simulink model "Three_Phase_Controlled"  (R2025b)
settings: Solver=VariableStepAuto  StartTime=0.0  StopTime=10.0  MaxStep=1e-4  RelTol=1e-3
libraries: nesl_utility x15, ee_lib x14, fl_lib x10
settings Model: Creator=USER  LastModifiedBy=USER

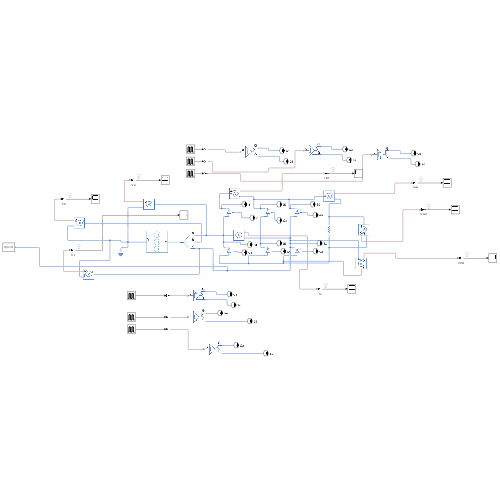
[thumbnail: Simulink's stored preview of the top-level diagram]
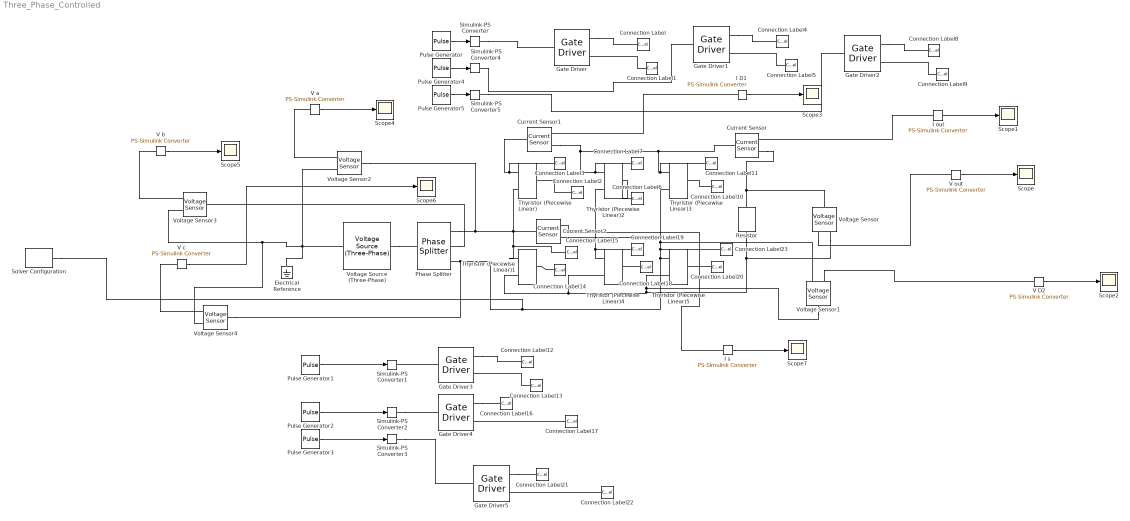
== system Three_Phase_Controlled ==
  Connection Label : ConnectionLabel  Label=G1
  Connection Label1 : ConnectionLabel  Label=S1
  Connection Label10 : ConnectionLabel  Label=G5
  Connection Label11 : ConnectionLabel  Label=S5
  Connection Label12 : ConnectionLabel  Label=G4
  Connection Label13 : ConnectionLabel  Label=S4
  Connection Label14 : ConnectionLabel  Label=G4
  Connection Label15 : ConnectionLabel  Label=S4
  Connection Label16 : ConnectionLabel  Label=G6
  Connection Label17 : ConnectionLabel  Label=S6
  Connection Label18 : ConnectionLabel  Label=G6
  Connection Label19 : ConnectionLabel  Label=S6
  Connection Label2 : ConnectionLabel  Label=G1
  Connection Label20 : ConnectionLabel  Label=G2
  Connection Label21 : ConnectionLabel  Label=G2
  Connection Label22 : ConnectionLabel  Label=S2
  Connection Label23 : ConnectionLabel  Label=S2
  Connection Label3 : ConnectionLabel  Label=S1
  Connection Label4 : ConnectionLabel  Label=G3
  Connection Label5 : ConnectionLabel  Label=S3
  Connection Label6 : ConnectionLabel  Label=G3
  Connection Label7 : ConnectionLabel  Label=S3
  Connection Label8 : ConnectionLabel  Label=G5
  Connection Label9 : ConnectionLabel  Label=S5
  Current Sensor : fl_lib/Electrical/Electrical Sensors/Current Sensor
  Current Sensor1 : fl_lib/Electrical/Electrical Sensors/Current Sensor
  Current Sensor2 : fl_lib/Electrical/Electrical Sensors/Current Sensor
  Electrical Reference : fl_lib/Electrical/Electrical Elements/Electrical Reference
  Gate Driver{,1..5} (6 alike) : ee_lib/Semiconductors & Converters/Gate Driver  port_option=ee.enum.controlport.ps  uHigh=2.0 V  uLow=0.8 V  uHighValue=0.7  uLowValue=0.3  vHigh=15 V  vLow=0 V  tHigh=50 ns  tLow=50 ns  parameterization=ee.enum.semiconductors.gateDriverParam.outputImpedance  rHigh=2 Ohm  rLow=2 Ohm  tRise=20 ns  tFall=20 ns  cLoad=10 nF  ZonTime_specify=off  ZonTime_priority=None  ZonTime=0 s  ZoffTime_specify=off  ZoffTime_priority=None  ZoffTime=0 s
      settings: InternalSimscapePortConfiguration="{\"Bottom\":[],\"Left\":[{\"id\":\"u\",\"label\":\"u\",\"type\":\"input\"}],\"Right\":[{\"id\":\"G\",\"label\":\"G\",\"type\":\"foundation.electrical.electrical\"},{\"id\":\"S\",\"label\":\"S\",\"type\":\"foundation.electrical.electrical\"}],\"Top\":[]}"
  I D1 : nesl_utility/PS-Simulink Converter  PhysicalDomain=network_engine_domain  SubClassName=ps_output  LeftPortType=input  RightPortType=output  PseudoPeriodic=off  Frequencies=[]  VectorFormat=inherit  Unit=inherit  AffineConversion=off
  I out : nesl_utility/PS-Simulink Converter  PhysicalDomain=network_engine_domain  SubClassName=ps_output  LeftPortType=input  RightPortType=output  PseudoPeriodic=off  Frequencies=[]  VectorFormat=inherit  Unit=inherit  AffineConversion=off
  I s : nesl_utility/PS-Simulink Converter  PhysicalDomain=network_engine_domain  SubClassName=ps_output  LeftPortType=input  RightPortType=output  PseudoPeriodic=off  Frequencies=[]  VectorFormat=inherit  Unit=inherit  AffineConversion=off
  Phase Splitter : ee_lib/Connectors & References/Phase Splitter
  Pulse Generator : DiscretePulseGenerator  PulseType=Time based  Period=1/50  PulseWidth=33.3  PhaseDelay=(30+30) * 0.02 / 360
  Pulse Generator1 : DiscretePulseGenerator  PulseType=Time based  Period=1/50  PulseWidth=33.3  PhaseDelay="(30 +  210) * 0.02 / 360"
  Pulse Generator2 : DiscretePulseGenerator  PulseType=Time based  Period=1/50  PulseWidth=33.3  PhaseDelay=(30+330) * 0.02 / 360
  Pulse Generator3 : DiscretePulseGenerator  PulseType=Time based  Period=1/50  PulseWidth=33.3  PhaseDelay=( 30+90) * 0.02 / 360
  Pulse Generator4 : DiscretePulseGenerator  PulseType=Time based  Period=1/50  PulseWidth=33.3  PhaseDelay=(30+150) * 0.02 / 360
  Pulse Generator5 : DiscretePulseGenerator  PulseType=Time based  Period=1/50  PulseWidth=33.3  PhaseDelay=( 30+270) * 0.02 / 360
  Resistor : fl_lib/Electrical/Electrical Elements/Resistor  R=200 Ohm  i_specify=off  i_priority=None  i=0 A  i_nominal_specify=off  i_nominal_value=1  i_nominal_unit=A  v_specify=off  v_priority=None  v=0 V  v_nominal_specify=off  v_nominal_value=1  v_nominal_unit=V
  Scope{,1..7} (8 alike) : Scope
      Scope settings: ActiveDisplayYMinimum=-8.8817841970012523E-15  ActiveDisplayYMaximum=8.8817841970012523E-15
      Scope1 settings: ActiveDisplayYMinimum=-6.5511151231257829E-17  ActiveDisplayYMaximum=3.7755575615628916E-17
      Scope2 settings: ActiveDisplayYMinimum=-1  ActiveDisplayYMaximum=1  DataLoggingVariableName=ScopeData2
      Scope3 settings: DataLoggingVariableName=ScopeData3
      Scope4 settings: DataLoggingVariableName=ScopeData4
      Scope5 settings: ActiveDisplayYMinimum=-1  ActiveDisplayYMaximum=1  DataLoggingVariableName=ScopeData5
      Scope6 settings: DataLoggingVariableName=ScopeData6
      Scope7 settings: DataLoggingVariableName=ScopeData7
  Simulink-PS Converter{,1..5} (6 alike) : nesl_utility/Simulink-PS Converter  PhysicalDomain=network_engine_domain  SubClassName=ps_input  LeftPortType=input  RightPortType=output  PseudoPeriodic=off  Frequencies=[]  NoiseDistribution=none  NoiseParameters=[]  Unit=V  AffineConversion=off  FilteringAndDerivatives=provide  SimscapeFilterOrder=1  InputFilterTimeConstant=0.001  UdotUserProvided=0
  Solver Configuration : nesl_utility/Solver Configuration  PhysicalDomain=network_engine_domain  SubClassName=solver  LeftPortType=input  RightPortType=generic  Tones=[]  Harmonics=[]  SimulateNoise=off  Profile=off  UseLocalSampling=off  EnableSwitchedLinearOptims=on  FrequencyDomain=off  UseCCode=off  RelTol=0.001  AbsTol=0.001  MinStep=1e-09  ToWorkspace=off  RevertToSquareIcSolve=off  NumHomotopyIterations=100  PhasorMode=off  PhasorModeNumHarmonics=1  ConsistencySolver=NEWTON_XTOL_AFTER_FTOL  IndexReductionMethod=DerivativeReplacement  DoDC=on  ResidualTolerance=1e-09  ConsistencyTolSource=GLOBAL  ConsistencyAbsTol=0.001  ConsistencyRelTol=0.001  ConsistencyTolFactor=0.001  UseLocalSolver=off  LocalSolverChoice=NE_BACKWARD_EULER_ADVANCER  ResolveIndetEquations=on  FunctionEvalNumThread=1  LocalSolverSampleTime=0.001  DoFixedCost=off  MaxNonlinIter=3  MaxModeIter=2  ComputeImpulses=off  ImpulseIterations=2  LinearAlgebra=auto  LinearAlgebraNumThread=0  EquationFormulation=NE_TIME_EF  DelaysMemoryBudget=1024  AutomaticFiltering=on  FilteringTimeConstant=0.001  PartitionStorageMethod=AS_NEEDED  PartitionMemoryBudget=1024  PartitionMethod=ROBUST  MultibodyUseLocalSolver=off  MultibodyLocalSolverChoice=ODE1  MultibodyLocalSolverSampleTime=0.001
  Thyristor (Piecewise Linear){,1..5} (6 alike) : ee_lib/Semiconductors & Converters/Thyristor (Piecewise Linear)  port_option=ee.enum.controlport.elec  Vf=0.8 V  Ron=0.001 Ohm  Goff=1e-5 1/Ohm  Vgt=6 V  Ih=1 A  diode_param=ee.enum.semiconductors.protectionDiode.external  diode_Vf=0.8 V  diode_Ron=0.001 Ohm  diode_Goff=1e-5 1/Ohm  diode_C=50e-9 F  diode_iRM=-235 A  diode_iF=300 A  diode_idot=-50 A/us  diode_trr_param=ee.enum.converters.diodetrr.trr_factor  diode_trr_factor=3  diode_trr=15 us  diode_Qrr=1500 s*uA  iak_specify=off  iak_priority=None  iak=0 A  iak_nominal_specify=off  iak_nominal_value=1  iak_nominal_unit=A  vak_specify=off  vak_priority=None  vak=0 V  vak_nominal_specify=off  vak_nominal_value=1  vak_nominal_unit=V  vgk_specify=off  vgk_priority=None  vgk=0 V  vgk_nominal_specify=off  vgk_nominal_value=1  vgk_nominal_unit=V  thermal_loss_option=ee.enum.converters.thermalLossOption.constantvalues  Von_data=[0, .1, .6, .8, 1, 1.3, 1.6, 2, 2.4; 0, .1, .7, 1, 1.2, 1.5, 1.9, 2.4, 2.8] V  Tj=[298.15, 398.15] K  Iout_data=[0, .1, 1, 5, 10, 20, 40, 70, 100] A  Eon_data=[0, .0024, .024, .12, .2, .48, 1.04, 2.16, 3.24; 0, .003, .03, .15, .25, .6, 1.3, 2.7, 4.05] * 1e-3 J  Tj_loss=[298.15, 398.15] K  Iout_data_loss=[0, .1, 1, 5, 10, 20, 40, 70, 100] A  Eon_scalar=22.86e-3 J  Eoff_natural_commutation=10e-3 J  Voff=300 V  Iout_scalar=600 A  onCurrentMeasDelay=1e-4 s  diodeModelType=ee.enum.converters.diodeModelType.pwl  diodeTableType=ee.enum.diode.tableType.IfMat  diode_IfMat=[.07, .12, .19, 1.75, 4.24, 7.32, 11.2; .16, .3, .72, 2.14, 4.02, 6.35, 9.12] A  diode_VfMat=[.9, 1.15, 1.25, 1.5, 1.75, 2.17, 2.6, 2.85; .58, .68, .75, 1.1, 1.38, 1.77, 2.27, 2.7] V  diode_TjVec=[25, 125] degC  diode_VfVec=[.5, .7, .9, 1.3, 1.7, 2.1, 2.5] V  diode_IfVec=[.1, .2, .5, 1, 2, 4, 7, 10] A  diode_rec_loss_model=ee.enum.diode.reverseRecoveryModel.fixed  diode_ErecVal=0 J  diode_scaleWithIandV=true  diode_ErecMat=zeros(2, 3) J  diode_TjrecVec=[298.15, 398.15] K  diode_IfrecVec=[.1, 1, 10] A  diode_IrecVal=10 A  diode_VrecVal=10 V  diode_tFilter=1 / 1000 / 100 s  thermal_network_parameterization=ee.enum.thermalNetworkTopology.external  Rth=[.08, .5] K/W  Rth_Cauer=[.08, .1, .5] K/W  Rth_Foster=[.08, .14, .22, .16] K/W  thermal_mass_parameterization=ee.enum.thermalNetwork.timeconstant  thermal_mass=[.01, .5] J/K  thermal_mass_Cauer=[.01, .1, .5] J/K  thermal_mass_Foster=[.001, .005, .05, .5] J/K  thermal_time_constant=[.001, .2] s  thermal_time_constant_Cauer=[.001, .1, .2] s  thermal_time_constant_Foster=[7e-05, .0007, .01, .08] s  thermal_mass_initial_temperatures=[25, 25] degC  thermal_mass_initial_temperatures_Cauer=[25, 25, 25] degC  junction_thermal_mass=0.01 J/K  Tvec_initial_Foster=[25, 25, 25, 25] degC  junction_temperature_specify=off  junction_temperature_priority=None  junction_temperature=25 degC  junction_temperature_nominal_specify=off  junction_temperature_nominal_value=1  junction_temperature_nominal_unit=degC  Qj_specify=off  Qj_priority=None  Qj=0 W  Qj_nominal_specify=off  Qj_nominal_value=1  Qj_nominal_unit=W  accumulatedSwitchingLosses_specify=off  accumulatedSwitchingLosses_priority=None  accumulatedSwitchingLosses=0 J
      settings: InternalSimscapePortConfiguration="{\"Bottom\":[],\"Left\":[{\"id\":\"G_elec\",\"label\":\"\",\"type\":\"foundation.electrical.electrical\"}],\"Right\":[{\"id\":\"A\",\"label\":\"\",\"type\":\"foundation.electrical.electrical\"},{\"id\":\"K\",\"label\":\"\",\"type\":\"foundation.electrical.electrical\"}],\"Top\":[]}"
  V D2 : nesl_utility/PS-Simulink Converter  PhysicalDomain=network_engine_domain  SubClassName=ps_output  LeftPortType=input  RightPortType=output  PseudoPeriodic=off  Frequencies=[]  VectorFormat=inherit  Unit=inherit  AffineConversion=off
  V a : nesl_utility/PS-Simulink Converter  PhysicalDomain=network_engine_domain  SubClassName=ps_output  LeftPortType=input  RightPortType=output  PseudoPeriodic=off  Frequencies=[]  VectorFormat=inherit  Unit=inherit  AffineConversion=off
  V b : nesl_utility/PS-Simulink Converter  PhysicalDomain=network_engine_domain  SubClassName=ps_output  LeftPortType=input  RightPortType=output  PseudoPeriodic=off  Frequencies=[]  VectorFormat=inherit  Unit=inherit  AffineConversion=off
  V c : nesl_utility/PS-Simulink Converter  PhysicalDomain=network_engine_domain  SubClassName=ps_output  LeftPortType=input  RightPortType=output  PseudoPeriodic=off  Frequencies=[]  VectorFormat=inherit  Unit=inherit  AffineConversion=off
  V out : nesl_utility/PS-Simulink Converter  PhysicalDomain=network_engine_domain  SubClassName=ps_output  LeftPortType=input  RightPortType=output  PseudoPeriodic=off  Frequencies=[]  VectorFormat=inherit  Unit=inherit  AffineConversion=off
  Voltage Source (Three-Phase) : ee_lib/Sources/Voltage Source (Three-Phase)  vline_rms=45 * sqrt(3) V  shift=0 deg  freq=50 Hz  impedance_option=1  SShortCircuit=1e6 A*V  XR=15  R=0.01 Ohm  L=3.97e-4 H  harmonic_option=0  harmonic_orders=[5, 7, 11, 13]  harmonic_ratios=[.1, .1, .1, .1]  G_parasitic=0 1/Ohm  I_specify=off  I_priority=None  I=[0, 0, 0] A  I_nominal_specify=off  I_nominal_value=1  I_nominal_unit=A
  Voltage Sensor{,1..4} (5 alike) : fl_lib/Electrical/Electrical Sensors/Voltage Sensor
  wires:
  Pulse Generator/1 -> Simulink-PS Converter/1
  Pulse Generator1/1 -> Simulink-PS Converter1/1
  Pulse Generator2/1 -> Simulink-PS Converter2/1
  Pulse Generator3/1 -> Simulink-PS Converter3/1
  Pulse Generator4/1 -> Simulink-PS Converter4/1
  Pulse Generator5/1 -> Simulink-PS Converter5/1
  V out/1 -> Scope/1
  I out/1 -> Scope1/1
  V D2/1 -> Scope2/1
  I D1/1 -> Scope3/1
  V a/1 -> Scope4/1
  V b/1 -> Scope5/1
  V c/1 -> Scope6/1
  I s/1 -> Scope7/1
  connections:
  Voltage Source (Three-Phase)/LConn1 -- Voltage Sensor4/RConn2 -- Voltage Sensor3/RConn2 -- Electrical Reference/LConn1 -- Voltage Sensor2/RConn2
  Thyristor (Piecewise Linear)1/RConn2 -- Connection Label15/LConn1 -- Current Sensor2/LConn1 -- Voltage Sensor2/LConn1 -- Phase Splitter/RConn1 -- Thyristor (Piecewise Linear)/RConn1
  Thyristor (Piecewise Linear)3/RConn2 -- Connection Label11/LConn1 -- Connection Label7/LConn1 -- Thyristor (Piecewise Linear)2/RConn2 -- Current Sensor1/RConn2 -- Current Sensor/LConn1
  Thyristor (Piecewise Linear)1/RConn1 -- Voltage Sensor1/LConn1 -- Thyristor (Piecewise Linear)5/RConn1 -- Voltage Sensor/RConn2 -- Resistor/RConn1 -- Thyristor (Piecewise Linear)4/RConn1
  Thyristor (Piecewise Linear)4/RConn2 -- Connection Label19/LConn1 -- Thyristor (Piecewise Linear)2/RConn1
  Thyristor (Piecewise Linear)5/RConn2 -- Solver Configuration/RConn1 -- Voltage Sensor4/LConn1 -- Phase Splitter/RConn3 -- Connection Label23/LConn1 -- Current Sensor2/RConn2 -- Thyristor (Piecewise Linear)3/RConn1 -- Voltage Sensor1/RConn2
  Voltage Source (Three-Phase)/RConn1 -- Phase Splitter/LConn1
  Voltage Sensor/RConn1 -- V out/LConn1
  Resistor/LConn1 -- Current Sensor/RConn2 -- Voltage Sensor/LConn1
  I out/LConn1 -- Current Sensor/RConn1
  V D2/LConn1 -- Voltage Sensor1/RConn1
  Thyristor (Piecewise Linear)/RConn2 -- Connection Label3/LConn1 -- Current Sensor1/LConn1
  I D1/LConn1 -- Current Sensor1/RConn1
  V a/LConn1 -- Voltage Sensor2/RConn1
  V b/LConn1 -- Voltage Sensor3/RConn1
  V c/LConn1 -- Voltage Sensor4/RConn1
  Phase Splitter/RConn2 -- Voltage Sensor3/LConn1
  I s/LConn1 -- Current Sensor2/RConn1
  Simulink-PS Converter/RConn1 -- Gate Driver/LConn1
  Gate Driver/RConn1 -- Connection Label/LConn1
  Connection Label1/LConn1 -- Gate Driver/RConn2
  Connection Label2/LConn1 -- Thyristor (Piecewise Linear)/LConn1
  Connection Label5/LConn1 -- Gate Driver1/RConn2
  Gate Driver1/RConn1 -- Connection Label4/LConn1
  Simulink-PS Converter4/RConn1 -- Gate Driver1/LConn1
  Connection Label6/LConn1 -- Thyristor (Piecewise Linear)2/LConn1
  Connection Label9/LConn1 -- Gate Driver2/RConn2
  Gate Driver2/RConn1 -- Connection Label8/LConn1
  Simulink-PS Converter5/RConn1 -- Gate Driver2/LConn1
  Connection Label10/LConn1 -- Thyristor (Piecewise Linear)3/LConn1
  Gate Driver3/RConn1 -- Connection Label12/LConn1
  Connection Label13/LConn1 -- Gate Driver3/RConn2
  Gate Driver3/LConn1 -- Simulink-PS Converter1/RConn1
  Connection Label14/LConn1 -- Thyristor (Piecewise Linear)1/LConn1
  Connection Label17/LConn1 -- Gate Driver4/RConn2
  Gate Driver4/RConn1 -- Connection Label16/LConn1
  Simulink-PS Converter2/RConn1 -- Gate Driver4/LConn1
  Connection Label18/LConn1 -- Thyristor (Piecewise Linear)4/LConn1
  Gate Driver5/RConn1 -- Connection Label21/LConn1
  Connection Label22/LConn1 -- Gate Driver5/RConn2
  Simulink-PS Converter3/RConn1 -- Gate Driver5/LConn1
  Connection Label20/LConn1 -- Thyristor (Piecewise Linear)5/LConn1
